simulink model "untitled"  (R2024b)
settings: Solver=VariableStepAuto  StartTime=0.0  StopTime=0.3  RelTol=1e-3
values from neighbouring files (symbols this model uses):
  A = [-Ra/La, -K/La; K/J,    0]    [lab.m]
  B = [1/La,  0; 0, -1/J]    [lab.m]
  C = [1, 0; 0, 1]    [lab.m]
  D = [0, 0; 0, 0]    [lab.m]
  ts = 0.001    [lab.m]
settings Model: Creator=rober  LastModifiedBy=rober

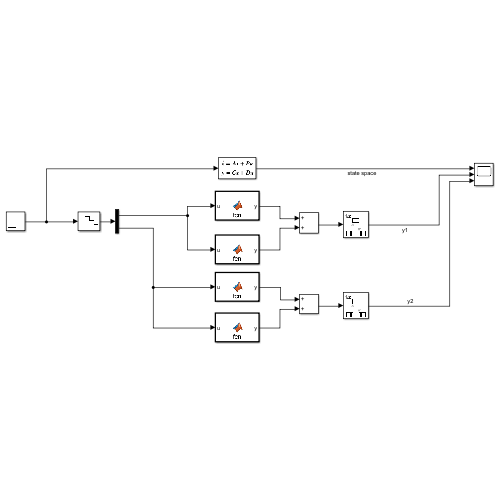
[thumbnail: Simulink's stored preview of the top-level diagram]
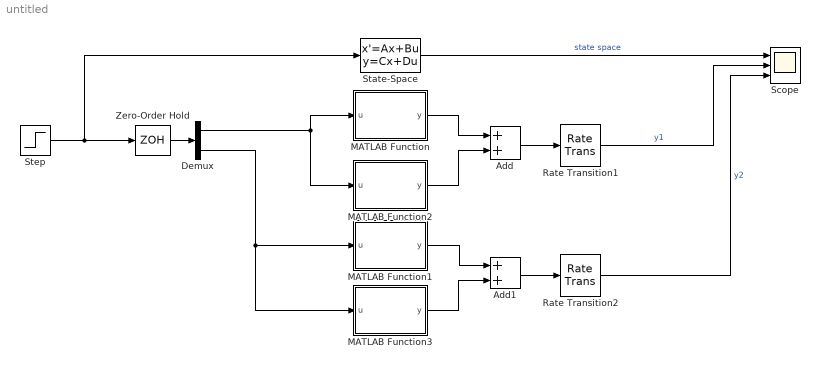
== system untitled ==
  Add : Sum
  Add1 : Sum
  Demux : Demux  Outputs=2
  MATLAB Function : MATLAB Function  TreatAsAtomicUnit=on
  MATLAB Function1 : MATLAB Function  TreatAsAtomicUnit=on
  MATLAB Function2 : MATLAB Function  TreatAsAtomicUnit=on
  MATLAB Function3 : MATLAB Function  TreatAsAtomicUnit=on
  Rate Transition1 : RateTransition
  Rate Transition2 : RateTransition
  Scope : Scope  NumInputPorts=3
  State-Space : StateSpace  A=A  B=B  C=C  D=D  InitialCondition=0
  Step : Step  Time=0  Before=[0, 0]  After=[25; 0]  SampleTime=ts
  Zero-Order Hold : ZeroOrderHold  SampleTime=ts
  wires:
  Step/1 -> State-Space/1, Zero-Order Hold/1
  Demux/1 -> MATLAB Function2/1(u), MATLAB Function/1(u)
  MATLAB Function/1(y) -> Add/1
  MATLAB Function1/1(y) -> Add1/1
  Add/1 -> Rate Transition1/1
  Rate Transition1/1 -> Scope/2  "y1"
  Demux/2 -> MATLAB Function1/1(u), MATLAB Function3/1(u)
  Rate Transition2/1 -> Scope/3  "y2"
  Add1/1 -> Rate Transition2/1
  Zero-Order Hold/1 -> Demux/1
  MATLAB Function3/1(y) -> Add1/2
  State-Space/1 -> Scope/1  "state space"
  MATLAB Function2/1(y) -> Add/2

== matlab function untitled/MATLAB Function ==
  data: u input; y output
function y = fcn(u)

persistent y1 y2 u1 u2;

if isempty(y1)
    y1 = 0;
end

if isempty(y2)
    y2 = 0;
end

if isempty(u1)
    u1 = 0;
end

if isempty(u2)
    u2 = 0;
end

a = 0.346;
b = -0.346;
c = -1.41;
d = 0.4421;

y = - c * y1 - d * y2 + a * u1 + b * u2;

u2 = u1;
u1 = u;
y2 = y1;
y1 = y;

== matlab function untitled/MATLAB Function2 ==
  data: y output; u input
function y = fcn(u)

persistent y1 y2 u1 u2;

if isempty(y1)
    y1 = 0;
end

if isempty(y2)
    y2 = 0;
end

if isempty(u1)
    u1 = 0;
end

if isempty(u2)
    u2 = 0;
end


a = 0.2791;
b = 0.2128;
c = -1.41;
d = 0.4421;

y = - c * y1 - d * y2 + a * u1 + b * u2;

u2 = u1;
u1 = u;
y2 = y1;
y1 = y;

== matlab function untitled/MATLAB Function3 ==
  data: u input; y output
function y = fcn(u)

persistent y1 y2 u1 u2;

if isempty(y1)
    y1 = 0;
end

if isempty(y2)
    y2 = 0;
end

if isempty(u1)
    u1 = 0;
end

if isempty(u2)
    u2 = 0;
end


a = -21.65;
b = 9.537;
c = -1.41;
d = 0.4421;

y = - c * y1 - d * y2 + a * u1 + b * u2;

u2 = u1;
u1 = u;
y2 = y1;
y1 = y;

== matlab function untitled/MATLAB Function1 ==
  data: y output; u input
function y = fcn(u)

persistent y1 y2 u1 u2;

if isempty(y1)
    y1 = 0;
end

if isempty(y2)
    y2 = 0;
end

if isempty(u1)
    u1 = 0;
end

if isempty(u2)
    u2 = 0;
end


a = 0.2791;
b = 0.2128;
c = -1.41;
d = 0.4421;

y = - c * y1 - d * y2 + a * u1 + b * u2;

u2 = u1;
u1 = u;
y2 = y1;
y1 = y;
